simulink model "part4_energy_and_money"  (R2026a)
settings: Solver=ode1  StopTime=24.0  FixedStep=0.001
libraries: simulink x5
settings Model: Creator=HAKAN SARI  LastModifiedBy=HAKAN SARI

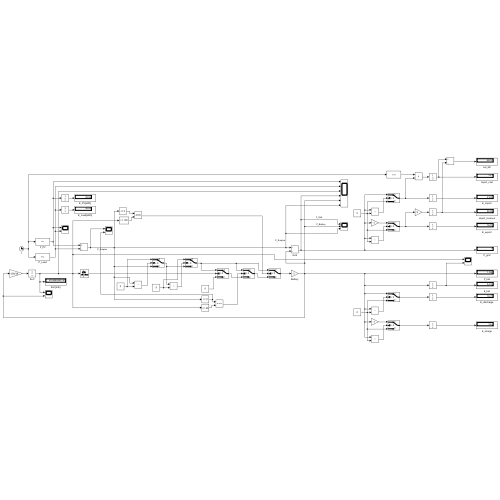
[thumbnail: Simulink's stored preview of the top-level diagram]
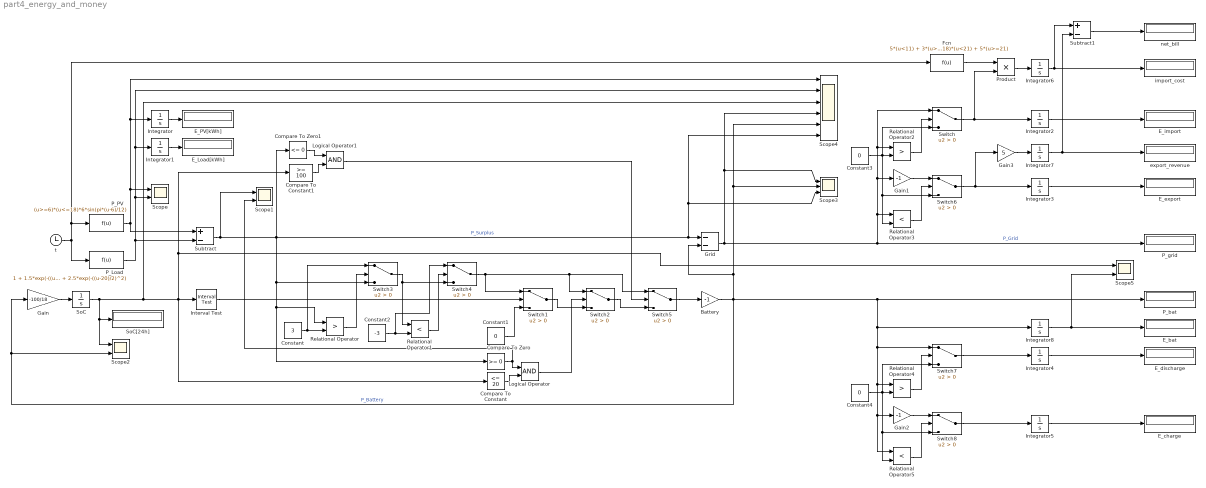
== system part4_energy_and_money ==
  Battery : Gain  Gain=-1
  Compare To Constant : simulink/Logic and Bit Operations/Compare To Constant  relop=<=  const=20  OutDataTypeStr=boolean
  Compare To Constant1 : simulink/Logic and Bit Operations/Compare To Constant  relop=>=  const=100  OutDataTypeStr=boolean
  Compare To Zero : simulink/Logic and Bit Operations/Compare To Zero  relop=>=  OutDataTypeStr=boolean
  Compare To Zero1 : simulink/Logic and Bit Operations/Compare To Zero  relop=<=  OutDataTypeStr=boolean
  Constant : Constant  Value=3
  Constant1 : Constant  Value=0
  Constant2 : Constant  Value=-3
  Constant3 : Constant  Value=0
  Constant4 : Constant  Value=0
  E_Load[kWh] : Display
  E_PV[kWh] : Display
  E_bat : Display
  E_charge : Display
  E_discharge : Display
  E_export : Display
  E_import : Display
  Fcn : Fcn  Expr=5*(u<11) + 3*(u>=11)*(u<18) + 10*(u>=18)*(u<21) + 5*(u>=21)
  Gain : Gain  Gain=-100/18
  Gain1 : Gain  Gain=-1
  Gain2 : Gain  Gain=-1
  Gain3 : Gain  Gain=5
  Grid : Sum  Inputs=--
  Integrator{,1..8} (9 alike) : Integrator
  Interval Test : simulink/Logic and Bit Operations/Interval Test  IntervalClosedRight=off  uplimit=100  IntervalClosedLeft=off  lowlimit=20  OutDataTypeStr=boolean
  Logical Operator : Logic  AllPortsSameDT=off  OutDataTypeStr=boolean
  Logical Operator1 : Logic  AllPortsSameDT=off  OutDataTypeStr=boolean
  P_Load : Fcn  Expr=1 + 1.5*exp(-((u-8)/1.5)^2) + 2.5*exp(-((u-20)/2)^2)
  P_PV : Fcn  Expr=(u>=6)*(u<=18)*6*sin(pi*(u-6)/12)
  P_bat : Display
  P_grid : Display
  Product : Product
  Relational Operator : RelationalOperator  Operator=>  OutDataTypeStr=boolean  RndMeth=Simplest  InputSameDT=off
  Relational Operator1 : RelationalOperator  Operator=<  OutDataTypeStr=boolean  RndMeth=Simplest  InputSameDT=off
  Relational Operator2 : RelationalOperator  Operator=>  OutDataTypeStr=boolean  RndMeth=Simplest  InputSameDT=off
  Relational Operator3 : RelationalOperator  Operator=<  OutDataTypeStr=boolean  RndMeth=Simplest  InputSameDT=off
  Relational Operator4 : RelationalOperator  Operator=>  OutDataTypeStr=boolean  RndMeth=Simplest  InputSameDT=off
  Relational Operator5 : RelationalOperator  Operator=<  OutDataTypeStr=boolean  RndMeth=Simplest  InputSameDT=off
  Scope{,1..2,5} (4 alike) : Scope  NumInputPorts=2
      Scope settings: MaximizeAxes=On  ActiveDisplayYMinimum=-1  ActiveDisplayYMaximum=1
      Scope1 settings: ActiveDisplayYMinimum=-4.5623497463789127  ActiveDisplayYMaximum=6.0611477174102166
      Scope2 settings: ActiveDisplayYMinimum=9.9405360115103285  ActiveDisplayYMaximum=110.16983442047547  DataLoggingVariableName=ScopeData2
      Scope5 settings: MaximizeAxes=On  ActiveDisplayYMinimum=9.9969361474422715  ActiveDisplayYMaximum=110.00136512238805  DataLoggingVariableName=ScopeData5
  Scope3 : Scope  NumInputPorts=3
      settings: MaximizeAxes=On  ActiveDisplayYMinimum=-5.3458837539306616  ActiveDisplayYMaximum=1.9867870538912946  DataLoggingVariableName=ScopeData3
  Scope4 : Scope  NumInputPorts=6
      settings: MaximizeAxes=On  ActiveDisplayString=6  ActiveDisplayYMinimum=-4.5623497463789127  ActiveDisplayYMaximum=6.0611477174102166  DataLoggingVariableName=ScopeData4
  SoC : Integrator  InitialCondition=50
  SoC[24h] : Display
  Subtract : Sum  Inputs=+-
  Subtract1 : Sum  Inputs=+-
  Switch{,1..8} (9 alike) : Switch  Criteria=u2 > Threshold  SaturateOnIntegerOverflow=off  InputSameDT=off
  export_revenue : Display
  import_cost : Display
  net_bill : Display
  t : Clock
  wires:
  P_PV/1 -> Scope4/1, Integrator/1, Scope/1, Subtract/1
  P_Load/1 -> Scope4/2, Integrator1/1, Scope/2, Subtract/2
  Subtract/1 -> Switch3/3, Compare To Zero/1, Relational Operator/1, Scope4/6, Scope3/3, Grid/1, Compare To Zero1/1, Scope1/1  "P_Surplus"
  SoC/1 -> SoC[24h]/1, Scope2/1, Scope4/3, Interval Test/1, Compare To Constant/1, Scope5/1, Compare To Constant1/1
  Interval Test/1 -> Switch1/2
  Constant1/1 -> Switch1/3
  Compare To Constant/1 -> Logical Operator/2
  Compare To Zero/1 -> Scope1/2, Logical Operator/1
  Logical Operator/1 -> Switch2/2
  Switch1/1 -> Switch2/3
  Compare To Zero1/1 -> Logical Operator1/1
  Compare To Constant1/1 -> Logical Operator1/2
  Switch5/1 -> Battery/1
  Logical Operator1/1 -> Switch5/2
  Switch2/1 -> Switch5/3
  t/1 -> Fcn/1, P_PV/1, P_Load/1
  Integrator/1 -> E_PV[kWh]/1
  Integrator1/1 -> E_Load[kWh]/1
  Gain/1 -> SoC/1
  Battery/1 -> Scope2/2, Gain/1, Integrator8/1, Relational Operator5/1, Gain2/1, Relational Operator4/1, Switch7/1, P_bat/1, Scope4/5, Scope3/2, Grid/2  "P_Battery"
  Constant/1 -> Relational Operator/2, Switch3/1
  Constant2/1 -> Relational Operator1/2, Switch4/1
  Relational Operator/1 -> Switch3/2
  Relational Operator1/1 -> Switch4/2
  Switch3/1 -> Switch4/3, Relational Operator1/1
  Switch4/1 -> Switch5/1, Switch2/1, Switch1/1
  Grid/1 -> Scope4/4, Scope3/1, P_grid/1, Relational Operator3/1, Switch/1, Relational Operator2/1, Gain1/1  "P_Grid"
  Constant3/1 -> Relational Operator3/2, Switch6/3, Switch/3, Relational Operator2/2
  Relational Operator2/1 -> Switch/2
  Switch/1 -> Product/2, Integrator2/1
  Integrator2/1 -> E_import/1
  Switch6/1 -> Gain3/1, Integrator3/1
  Relational Operator3/1 -> Switch6/2
  Integrator3/1 -> E_export/1
  Gain1/1 -> Switch6/1
  Gain2/1 -> Switch8/1
  Integrator5/1 -> E_charge/1
  Relational Operator5/1 -> Switch8/2
  Switch7/1 -> Integrator4/1
  Constant4/1 -> Relational Operator5/2, Switch8/3, Switch7/3, Relational Operator4/2
  Relational Operator4/1 -> Switch7/2
  Integrator4/1 -> E_discharge/1
  Switch8/1 -> Integrator5/1
  Fcn/1 -> Product/1
  Product/1 -> Integrator6/1
  Integrator6/1 -> Subtract1/1, import_cost/1
  Gain3/1 -> Integrator7/1
  Integrator7/1 -> Subtract1/2, export_revenue/1
  Subtract1/1 -> net_bill/1
  Integrator8/1 -> Scope5/2, E_bat/1
